simulink model "EV_BMS_SOC"  (R2024a)
settings: Solver=ode4  StartTime=0  StopTime=600  FixedStep=1  RelTol=1e-3
settings Model: Creator=KAPIL  LastModifiedBy=KAPIL

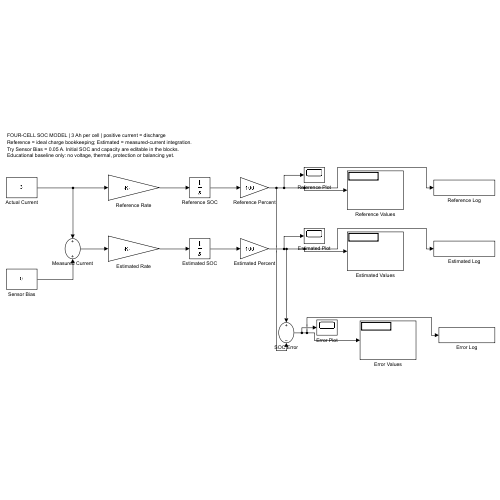
[thumbnail: Simulink's stored preview of the top-level diagram]
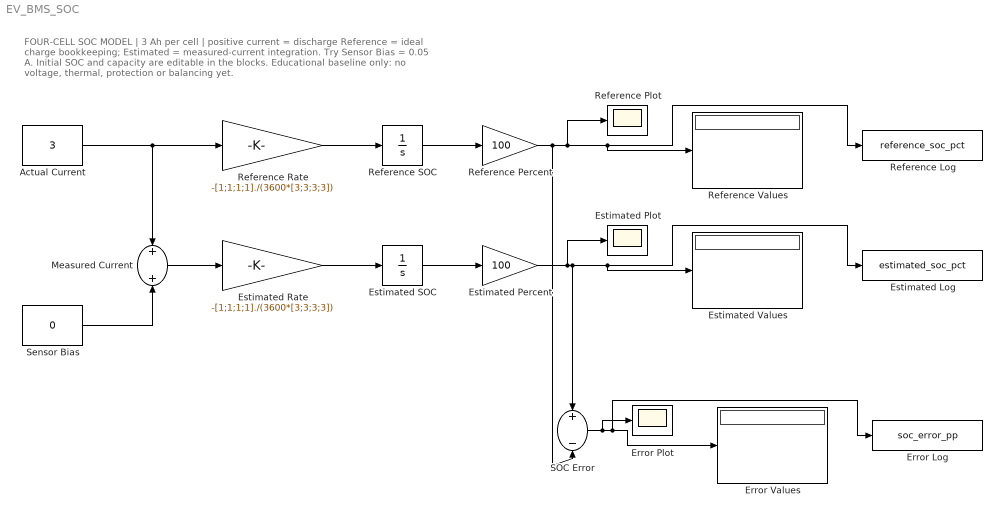
== system EV_BMS_SOC ==
  note: FOUR-CELL SOC MODEL | 3 Ah per cell | positive current = discharge
      | Reference = ideal charge bookkeeping; Estimated = measured-current integration.
      | Try Sensor Bias = 0.05 A. Initial SOC and capacity are editable in the blocks.
      | Educational baseline only: no voltage, thermal, protection or balancing yet.
  Actual Current : Constant  Value=3
  Error Log : ToWorkspace  VariableName=soc_error_pp  SaveFormat=Timeseries  SampleTime=-1
  Error Plot : Scope
  Error Values : Display
  Estimated Log : ToWorkspace  VariableName=estimated_soc_pct  SaveFormat=Timeseries  SampleTime=-1
  Estimated Percent : Gain  Gain=100
  Estimated Plot : Scope
  Estimated Rate : Gain  Gain=-[1;1;1;1]./(3600*[3;3;3;3])
  Estimated SOC : Integrator  InitialCondition=[0.80;0.78;0.76;0.74]
  Estimated Values : Display
  Measured Current : Sum
  Reference Log : ToWorkspace  VariableName=reference_soc_pct  SaveFormat=Timeseries  SampleTime=-1
  Reference Percent : Gain  Gain=100
  Reference Plot : Scope
  Reference Rate : Gain  Gain=-[1;1;1;1]./(3600*[3;3;3;3])
  Reference SOC : Integrator  InitialCondition=[0.80;0.78;0.76;0.74]
  Reference Values : Display
  SOC Error : Sum  Inputs=+-
  Sensor Bias : Constant  Value=0
  wires:
  Reference Rate/1 -> Reference SOC/1
  Reference SOC/1 -> Reference Percent/1
  Reference Percent/1 -> Reference Values/1, Reference Log/1, Reference Plot/1, SOC Error/2
  Estimated Rate/1 -> Estimated SOC/1
  Estimated SOC/1 -> Estimated Percent/1
  Estimated Percent/1 -> Estimated Values/1, Estimated Log/1, SOC Error/1, Estimated Plot/1
  Actual Current/1 -> Reference Rate/1, Measured Current/1
  Sensor Bias/1 -> Measured Current/2
  Measured Current/1 -> Estimated Rate/1
  SOC Error/1 -> Error Values/1, Error Log/1, Error Plot/1
